simulink model "proj3_optiona"  (R2024b)
settings: Solver=ode45  StartTime=0  StopTime=tf  FixedStep=1  MaxStep=10  RelTol=1e-10  AbsTol=1e-12
values from neighbouring files (symbols this model uses):
  a_L = 8000    [proj3a_main.m]
  e_L = 0.05    [proj3a_main.m]
  leader0 = [Lr0;Lv0]    [proj3a_main.m]
  mu = 3.986e5    (= 398600)    [proj3a_main.m]
  x0 = [rel_pos;rel_vel]    [proj3a_main.m]
undefined symbols (not defined in the file or in its folder): lead_orb, leader_angV, leaderP, rel_dyn
settings Model: Creator=yjxu
settings DataIOCC: SaveOutput=off

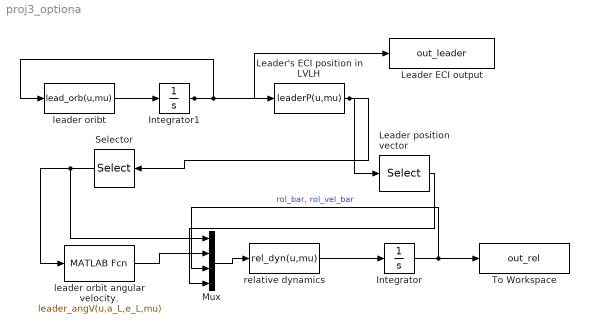
== system proj3_optiona ==
  Integrator : Integrator  InitialCondition=x0
  Integrator1 : Integrator  InitialCondition=leader0
  Leader ECI output : ToWorkspace  VariableName=out_leader  SaveFormat=Timeseries  SampleTime=-1
  Leader position vector : Selector  InputPortWidth=4  IndexOptions=Index vector (dialog)  Indices=[1 2 3]  OutputSizes=1
  Leader's ECI position in LVLH : MATLABFcn  MATLABFcn=leaderP(u,mu)  OutputDimensions=4
  Mux : Mux  Inputs=[1,2,6,3]
  Selector : Selector  InputPortWidth=4  IndexOptions=Index vector (dialog)  Indices=4  OutputSizes=1,1,1,1
  To Workspace : ToWorkspace  VariableName=out_rel  SaveFormat=Timeseries  SampleTime=-1
  leader orbit angular velocity. : MATLABFcn  MATLABFcn=leader_angV(u,a_L,e_L,mu)  OutputDimensions=2
  leader oribt : MATLABFcn  MATLABFcn=lead_orb(u,mu)  OutputDimensions=6
  relative dynamics : MATLABFcn  MATLABFcn=rel_dyn(u,mu)  OutputDimensions=6
  wires:
  relative dynamics/1 -> Integrator/1
  leader oribt/1 -> Integrator1/1
  Integrator1/1 -> Leader's ECI position in LVLH/1, leader oribt/1, Leader ECI output/1
  Mux/1 -> relative dynamics/1
  Integrator/1 -> To Workspace/1, Mux/3  "rol_bar, rol_vel_bar"
  leader orbit angular velocity./1 -> Mux/2
  Leader's ECI position in LVLH/1 -> Selector/1, Leader position vector/1
  Selector/1 -> leader orbit angular velocity./1, Mux/1
  Leader position vector/1 -> Mux/4
